simulink model "BEV_Thermal_Management"  (R2025a)
settings: Solver=ode23t  StartTime=0  StopTime=765  MaxStep=5  RelTol=1e-3  AbsTol=1e-3
model workspace: external: MATLAB File BEV_Thermal_Management_param.m (data not in the file)
undefined symbols (not defined in the file): Battery, bulb, cabin_doors_conductivity, cabin_duct_area, cabin_glass_conductivity, cabin_roof_conductivity, cabin_T_init, chiller_area_primary, chiller_N_baffles, chiller_N_tubes, chiller_tube_D, chiller_tube_L, chiller_wall_conductivity, chiller_wall_thickness, compressor_rpm_LUT, condenser_air_area_flow, condenser_air_area_primary, condenser_W, condenser_wall_conductivity, condenser_wall_thickness, coolant_channel_D, coolant_pipe_area, coolant_pipe_D, coolant_T_init, coolant_tank_area, coolant_tank_volume, coolant_valve_D_ratio_max, coolant_valve_D_ratio_min, coolant_valve_displacement, coolant_valve_S_max, cycle, DCDC, Edrive, evaporator_air_area_flow, evaporator_air_area_primary, evaporator_W, evaporator_wall_conductivity, evaporator_wall_thickness, heater_max_power, ModuleType1, outlet, ptc_max_power, pump_speed_max, radiationReflectionShields, radiator_air_area_flow, radiator_air_area_primary, radiator_W, radiator_wall_conductivity, radiator_wall_thickness, refrigerant_alpha_init, refrigerant_pipe_D, transRatio
libraries: fl_lib x264, nesl_utility x91, SimscapeFluids_lib x22, sdl_lib x13, ee_lib x9, nesl_utility_internal x4, slpidlib x3, BatteryProtection x3, batt_lib x2, BatteryCurrentManagement x1, autolibsharedcommon x1, simulink x1
(part 7 of 9)

== system BEV_Thermal_Management/Chiller/SR4 ==
  Absolute Reference (2P) : fl_lib/Two-Phase Fluid/Elements/Absolute Reference (2P)
  Mass & Energy Flow Rate Sensor (2P) : fl_lib/Two-Phase Fluid/Sensors/Flow Rate Sensor (2P)  mass_flow_measure=true  volumetric_flow_measure=false  energy_flow_measure=true
      settings: InternalSimscapePortConfiguration="{\"Bottom\":[{\"id\":\"PHI\",\"label\":\"φ\",\"type\":\"output\"}],\"Left\":[{\"id\":\"A\",\"label\":\"A\",\"type\":\"foundation.two_phase_fluid.two_phase_fluid\"}],\"Right\":[{\"id\":\"B\",\"label\":\"B\",\"type\":\"foundation.two_phase_fluid.two_phase_fluid\"},{\"id\":\"M\",\"label\":\"M\",\"type\":\"output\"}],\"Top\":[]}"
  PS-Simulink Converter : nesl_utility/PS-Simulink Converter  PhysicalDomain=network_engine_domain  SubClassName=ps_output  LeftPortType=input  RightPortType=output  PseudoPeriodic=off  Frequencies=[]  VectorFormat=1-D array  Unit=W  AffineConversion=off
  PS-Simulink Converter1 : nesl_utility/PS-Simulink Converter  PhysicalDomain=network_engine_domain  SubClassName=ps_output  LeftPortType=input  RightPortType=output  PseudoPeriodic=off  Frequencies=[]  VectorFormat=1-D array  Unit=MPa  AffineConversion=off
  PS-Simulink Converter2 : nesl_utility/PS-Simulink Converter  PhysicalDomain=network_engine_domain  SubClassName=ps_output  LeftPortType=input  RightPortType=output  PseudoPeriodic=off  Frequencies=[]  VectorFormat=inherit  Unit=degC  AffineConversion=off
  Pressure & Internal Energy Sensor (2P) : fl_lib/Two-Phase Fluid/Sensors/Pressure, Temperature & Internal Energy Sensor (2P)  reference=foundation.enum.MeasurementReference.difference  pressure=true  pressure_spec=foundation.enum.PressureMeasementSpec.Absolute  temperature=false  internal_energy=true
      settings: InternalSimscapePortConfiguration="{\"Bottom\":[{\"id\":\"U\",\"label\":\"U\",\"type\":\"output\"}],\"Left\":[{\"id\":\"A\",\"label\":\"A\",\"type\":\"foundation.two_phase_fluid.two_phase_fluid\"}],\"Right\":[{\"id\":\"B\",\"label\":\"B\",\"type\":\"foundation.two_phase_fluid.two_phase_fluid\"},{\"id\":\"P\",\"label\":\"P\",\"type\":\"output\"}],\"Top\":[]}"
  Terminator : Terminator
  Thermodynamic Properties Sensor (2P)1 : fl_lib/Two-Phase Fluid/Sensors/Thermodynamic Properties Sensor (2P)  temperature=true  enthalpy=true  density=false  specific_volume=true  entropy=true
      settings: InternalSimscapePortConfiguration="{\"Bottom\":[{\"id\":\"V\",\"label\":\"v\",\"type\":\"output\"},{\"id\":\"S\",\"label\":\"s\",\"type\":\"output\"}],\"Left\":[{\"id\":\"A\",\"label\":\"A\",\"type\":\"foundation.two_phase_fluid.two_phase_fluid\"}],\"Right\":[{\"id\":\"T\",\"label\":\"T\",\"type\":\"output\"},{\"id\":\"H\",\"label\":\"h\",\"type\":\"output\"}],\"Top\":[]}"
  B : PMIOPort  Side=Left
  A : PMIOPort  Port=2  Side=Right
  tag scope: Phi_chiller_out=global, p_chiller=global
  wires:
  PS-Simulink Converter/1 -> [Phi_chiller_out]
  PS-Simulink Converter1/1 -> [p_chiller]
  PS-Simulink Converter2/1 -> Terminator/1  "tempRefChillOut"
  connections:
  B/RConn1 -- Mass & Energy Flow Rate Sensor (2P)/RConn1
  Mass & Energy Flow Rate Sensor (2P)/LConn1 -- Thermodynamic Properties Sensor (2P)1/LConn1 -- Pressure & Internal Energy Sensor (2P)/LConn1 -- A/RConn1
  Mass & Energy Flow Rate Sensor (2P)/RConn3 -- PS-Simulink Converter/LConn1
  Absolute Reference (2P)/LConn1 -- Pressure & Internal Energy Sensor (2P)/RConn1
  PS-Simulink Converter1/LConn1 -- Pressure & Internal Energy Sensor (2P)/RConn2
  PS-Simulink Converter2/LConn1 -- Thermodynamic Properties Sensor (2P)1/RConn1

== system BEV_Thermal_Management/Compressor/Power sensor ==
  MRR3 : fl_lib/Mechanical/Rotational Elements/Mechanical Rotational Reference
  Pump power : fl_lib/Physical Signals/Functions/PS Product
  Rotational Motion Sensor : fl_lib/Mechanical/Mechanical Sensors/Ideal Rotational Motion Sensor  reference=foundation.enum.MeasurementReference.difference  acceleration_port=false  velocity_port=true  position_port=true  wrap_angle=simscape.enum.onoff.off  offset=0 rad
  Torque Sensor : fl_lib/Mechanical/Mechanical Sensors/Ideal Torque Sensor
  A : PMIOPort  Side=Left
  P : PMIOPort  Port=2  Side=Left
  B : PMIOPort  Port=3  Side=Right
  connections:
  Torque Sensor/RConn2 -- Pump power/LConn1
  Torque Sensor/RConn1 -- B/RConn1
  Rotational Motion Sensor/LConn1 -- Torque Sensor/LConn1 -- A/RConn1
  Rotational Motion Sensor/RConn2 -- Pump power/LConn2
  MRR3/LConn1 -- Rotational Motion Sensor/RConn1
  Pump power/RConn1 -- P/RConn1

== system BEV_Thermal_Management/Condenser/Power sensor ==
  MRR3 : fl_lib/Mechanical/Rotational Elements/Mechanical Rotational Reference
  Pump power : fl_lib/Physical Signals/Functions/PS Product
  Rotational Motion Sensor : fl_lib/Mechanical/Mechanical Sensors/Ideal Rotational Motion Sensor  reference=foundation.enum.MeasurementReference.difference  acceleration_port=false  velocity_port=true  position_port=true  wrap_angle=simscape.enum.onoff.off  offset=0 rad
  Torque Sensor : fl_lib/Mechanical/Mechanical Sensors/Ideal Torque Sensor
  A : PMIOPort  Side=Left
  P : PMIOPort  Port=2  Side=Left
  B : PMIOPort  Port=3  Side=Right
  connections:
  Torque Sensor/RConn2 -- Pump power/LConn1
  Torque Sensor/RConn1 -- B/RConn1
  Rotational Motion Sensor/LConn1 -- Torque Sensor/LConn1 -- A/RConn1
  Rotational Motion Sensor/RConn2 -- Pump power/LConn2
  MRR3/LConn1 -- Rotational Motion Sensor/RConn1
  Pump power/RConn1 -- P/RConn1

== system BEV_Thermal_Management/Condenser/SR1 ==
  Absolute Reference (2P) : fl_lib/Two-Phase Fluid/Elements/Absolute Reference (2P)
  Mass & Energy Flow Rate Sensor (2P) : fl_lib/Two-Phase Fluid/Sensors/Flow Rate Sensor (2P)  mass_flow_measure=true  volumetric_flow_measure=false  energy_flow_measure=true
      settings: InternalSimscapePortConfiguration="{\"Bottom\":[{\"id\":\"PHI\",\"label\":\"φ\",\"type\":\"output\"}],\"Left\":[{\"id\":\"A\",\"label\":\"A\",\"type\":\"foundation.two_phase_fluid.two_phase_fluid\"}],\"Right\":[{\"id\":\"B\",\"label\":\"B\",\"type\":\"foundation.two_phase_fluid.two_phase_fluid\"},{\"id\":\"M\",\"label\":\"M\",\"type\":\"output\"}],\"Top\":[]}"
  PS-Simulink Converter : nesl_utility/PS-Simulink Converter  PhysicalDomain=network_engine_domain  SubClassName=ps_output  LeftPortType=input  RightPortType=output  PseudoPeriodic=off  Frequencies=[]  VectorFormat=1-D array  Unit=W  AffineConversion=off
  PS-Simulink Converter2 : nesl_utility/PS-Simulink Converter  PhysicalDomain=network_engine_domain  SubClassName=ps_output  LeftPortType=input  RightPortType=output  PseudoPeriodic=off  Frequencies=[]  VectorFormat=inherit  Unit=degC  AffineConversion=off
  Pressure & Internal Energy Sensor (2P) : fl_lib/Two-Phase Fluid/Sensors/Pressure, Temperature & Internal Energy Sensor (2P)  reference=foundation.enum.MeasurementReference.difference  pressure=true  pressure_spec=foundation.enum.PressureMeasementSpec.Absolute  temperature=false  internal_energy=true
      settings: InternalSimscapePortConfiguration="{\"Bottom\":[{\"id\":\"U\",\"label\":\"U\",\"type\":\"output\"}],\"Left\":[{\"id\":\"A\",\"label\":\"A\",\"type\":\"foundation.two_phase_fluid.two_phase_fluid\"}],\"Right\":[{\"id\":\"B\",\"label\":\"B\",\"type\":\"foundation.two_phase_fluid.two_phase_fluid\"},{\"id\":\"P\",\"label\":\"P\",\"type\":\"output\"}],\"Top\":[]}"
  Terminator : Terminator
  Thermodynamic Properties Sensor (2P) : fl_lib/Two-Phase Fluid/Sensors/Thermodynamic Properties Sensor (2P)  temperature=true  enthalpy=true  density=false  specific_volume=true  entropy=true
      settings: InternalSimscapePortConfiguration="{\"Bottom\":[{\"id\":\"V\",\"label\":\"v\",\"type\":\"output\"},{\"id\":\"S\",\"label\":\"s\",\"type\":\"output\"}],\"Left\":[{\"id\":\"A\",\"label\":\"A\",\"type\":\"foundation.two_phase_fluid.two_phase_fluid\"}],\"Right\":[{\"id\":\"T\",\"label\":\"T\",\"type\":\"output\"},{\"id\":\"H\",\"label\":\"h\",\"type\":\"output\"}],\"Top\":[]}"
  A : PMIOPort  Side=Left
  B : PMIOPort  Port=2  Side=Right
  tag scope: Phi_cond_in=global
  wires:
  PS-Simulink Converter/1 -> [Phi_cond_in]
  PS-Simulink Converter2/1 -> Terminator/1  "tempRefCondIn"
  connections:
  Mass & Energy Flow Rate Sensor (2P)/LConn1 -- Pressure & Internal Energy Sensor (2P)/LConn1 -- Thermodynamic Properties Sensor (2P)/LConn1 -- A/RConn1
  B/RConn1 -- Mass & Energy Flow Rate Sensor (2P)/RConn1
  PS-Simulink Converter/LConn1 -- Mass & Energy Flow Rate Sensor (2P)/RConn3
  Absolute Reference (2P)/LConn1 -- Pressure & Internal Energy Sensor (2P)/RConn1
  PS-Simulink Converter2/LConn1 -- Thermodynamic Properties Sensor (2P)/RConn1

== system BEV_Thermal_Management/Condenser/SR2 ==
  Absolute Reference (2P) : fl_lib/Two-Phase Fluid/Elements/Absolute Reference (2P)
  Mass & Energy Flow Rate Sensor (2P) : fl_lib/Two-Phase Fluid/Sensors/Flow Rate Sensor (2P)  mass_flow_measure=true  volumetric_flow_measure=false  energy_flow_measure=true
      settings: InternalSimscapePortConfiguration="{\"Bottom\":[{\"id\":\"PHI\",\"label\":\"φ\",\"type\":\"output\"}],\"Left\":[{\"id\":\"A\",\"label\":\"A\",\"type\":\"foundation.two_phase_fluid.two_phase_fluid\"}],\"Right\":[{\"id\":\"B\",\"label\":\"B\",\"type\":\"foundation.two_phase_fluid.two_phase_fluid\"},{\"id\":\"M\",\"label\":\"M\",\"type\":\"output\"}],\"Top\":[]}"
  PS-Simulink Converter : nesl_utility/PS-Simulink Converter  PhysicalDomain=network_engine_domain  SubClassName=ps_output  LeftPortType=input  RightPortType=output  PseudoPeriodic=off  Frequencies=[]  VectorFormat=1-D array  Unit=W  AffineConversion=off
  PS-Simulink Converter1 : nesl_utility/PS-Simulink Converter  PhysicalDomain=network_engine_domain  SubClassName=ps_output  LeftPortType=input  RightPortType=output  PseudoPeriodic=off  Frequencies=[]  VectorFormat=1-D array  Unit=MPa  AffineConversion=off
  PS-Simulink Converter2 : nesl_utility/PS-Simulink Converter  PhysicalDomain=network_engine_domain  SubClassName=ps_output  LeftPortType=input  RightPortType=output  PseudoPeriodic=off  Frequencies=[]  VectorFormat=inherit  Unit=degC  AffineConversion=off
  Pressure & Internal Energy Sensor (2P) : fl_lib/Two-Phase Fluid/Sensors/Pressure, Temperature & Internal Energy Sensor (2P)  reference=foundation.enum.MeasurementReference.difference  pressure=true  pressure_spec=foundation.enum.PressureMeasementSpec.Absolute  temperature=false  internal_energy=true
      settings: InternalSimscapePortConfiguration="{\"Bottom\":[{\"id\":\"U\",\"label\":\"U\",\"type\":\"output\"}],\"Left\":[{\"id\":\"A\",\"label\":\"A\",\"type\":\"foundation.two_phase_fluid.two_phase_fluid\"}],\"Right\":[{\"id\":\"B\",\"label\":\"B\",\"type\":\"foundation.two_phase_fluid.two_phase_fluid\"},{\"id\":\"P\",\"label\":\"P\",\"type\":\"output\"}],\"Top\":[]}"
  Terminator : Terminator
  Thermodynamic Properties Sensor (2P) : fl_lib/Two-Phase Fluid/Sensors/Thermodynamic Properties Sensor (2P)  temperature=true  enthalpy=true  density=false  specific_volume=true  entropy=true
      settings: InternalSimscapePortConfiguration="{\"Bottom\":[{\"id\":\"V\",\"label\":\"v\",\"type\":\"output\"},{\"id\":\"S\",\"label\":\"s\",\"type\":\"output\"}],\"Left\":[{\"id\":\"A\",\"label\":\"A\",\"type\":\"foundation.two_phase_fluid.two_phase_fluid\"}],\"Right\":[{\"id\":\"T\",\"label\":\"T\",\"type\":\"output\"},{\"id\":\"H\",\"label\":\"h\",\"type\":\"output\"}],\"Top\":[]}"
  A : PMIOPort  Side=Left
  B : PMIOPort  Port=2  Side=Right
  tag scope: Phi_cond_out=global, p_cond=global
  wires:
  PS-Simulink Converter/1 -> [Phi_cond_out]
  PS-Simulink Converter1/1 -> [p_cond]
  PS-Simulink Converter2/1 -> Terminator/1  "tempRefCondOut"
  connections:
  Mass & Energy Flow Rate Sensor (2P)/LConn1 -- Thermodynamic Properties Sensor (2P)/LConn1 -- Pressure & Internal Energy Sensor (2P)/LConn1 -- A/RConn1
  B/RConn1 -- Mass & Energy Flow Rate Sensor (2P)/RConn1
  PS-Simulink Converter/LConn1 -- Mass & Energy Flow Rate Sensor (2P)/RConn3
  Absolute Reference (2P)/LConn1 -- Pressure & Internal Energy Sensor (2P)/RConn1
  PS-Simulink Converter1/LConn1 -- Pressure & Internal Energy Sensor (2P)/RConn2
  PS-Simulink Converter2/LConn1 -- Thermodynamic Properties Sensor (2P)/RConn1

== system BEV_Thermal_Management/Condenser/Speed command ==
  Max Speed [rpm] : Gain  Gain=1100
  Transfer Fcn : TransferFcn  Denominator=[5 1]
  Out1 : Outport
  wires:
  Transfer Fcn/1 -> Max Speed [rpm]/1
  Max Speed [rpm]/1 -> Out1/1
  [cmd_fan] -> Transfer Fcn/1

== system BEV_Thermal_Management/Controls/Cabin Air Control ==
  note: if the outside temperature is higher then the setpoint temperature turn off the PTC
  T_cabin : Inport
  T_setpoint : Inport  Port=2
  T_env : Inport  Port=3
  T_ptc : Inport  Port=4
  Add : Sum  Inputs=-+
  Constant : Constant  Commented=on  Value=0
  Constant1 : Constant  Value=0
  Old cmd ptc : Terminator  Commented=on
  PID Controller : slpidlib/PID Controller  Controller=PI  Form=Ideal  TimeDomain=Continuous-time  UseExternalTs=off  SampleTime=-1  IntegratorMethod=Forward Euler  FilterMethod=Forward Euler  ControllerParametersSource=internal  P=1/50  I=1/150  UseKiTs=off  D=0  UseExternalDerivativeSource=off  N=100  UseFilter=on  TunerSelectOption=Transfer Function Based (PID Tuner App)  InitialConditionSource=internal  InitialConditionForIntegrator=0  InitialConditionForFilter=0  DifferentiatorICPrevScaledInput=0  ExternalReset=none  TrackingMode=off  Kt=1  LimitOutput=on  SatLimitsSource=internal  UpperSaturationLimit=1  LowerSaturationLimit=0  LinearizeAsGain=on  AntiWindupMode=back-calculation  Kb=1  LimitIntegrator=off  UpperIntegratorSaturationLimit=inf  LowerIntegratorSaturationLimit=-inf  POutMin=[]  POutMax=[]  IOutMin=[]  IOutMax=[]  DOutMin=[]  DOutMax=[]  NOutMin=[]  NOutMax=[]  SumOutMin=[]  SumOutMax=[]  SaturationOutMin=[]  SaturationOutMax=[]  PParamMin=[]  PParamMax=[]  IParamMin=[]  IParamMax=[]  DParamMin=[]  DParamMax=[]  NParamMin=[]  NParamMax=[]  KbParamMin=[]  KbParamMax=[]  KtParamMin=[]  KtParamMax=[]  KbOutMin=[]  KbOutMax=[]  KtOutMin=[]  KtOutMax=[]  IntegratorOutMin=[]  IntegratorOutMax=[]  FilterOutMin=[]  FilterOutMax=[]  SumI1OutMin=[]  SumI1OutMax=[]  SumI2OutMin=[]  SumI2OutMax=[]  SumI3OutMin=[]  SumI3OutMax=[]  SumI4OutMin=[]  SumI4OutMax=[]  SumDOutMin=[]  SumDOutMax=[]  DifferentiatorOutMin=[]  DifferentiatorOutMax=[]  FilterDiffOutCoefMin=[]  FilterDiffOutCoefMax=[]  ReciprocalOutMin=[]  ReciprocalOutMax=[]  SumDenOutMin=[]  SumDenOutMax=[]  SumNumOutMin=[]  SumNumOutMax=[]  DivideOutMin=[]  DivideOutMax=[]  UdiffTsProdOutMin=[]  UdiffTsProdOutMax=[]  NTsProdOutMin=[]  NTsProdOutMax=[]  UintegralTsProdOutMin=[]  UintegralTsProdOutMax=[]  UngainTsProdOutMin=[]  UngainTsProdOutMax=[]  ClampingZeroOutDataTypeStr=Inherit: Inherit via back propagation  ClampingZeroOutMin=[]  ClampingZeroOutMax=[]  FilterDenConstantOutDataTypeStr=Inherit: Inherit via back propagation  FilterDenConstantOutMin=[]  FilterDenConstantOutMax=[]  PCopyOutDataTypeStr=Inherit: Inherit via back propagation  PCopyOutMin=[]  PCopyOutMax=[]  NCopyOutDataTypeStr=Inherit: Inherit via back propagation  NCopyOutMin=[]  NCopyOutMax=[]  IntegratorContinuousStateAttributes=''  IntegratorStateMustResolveToSignalObject=off  IntegratorRTWStateStorageClass=Auto  FilterContinuousStateAttributes=''  FilterStateMustResolveToSignalObject=off  FilterRTWStateStorageClass=Auto  ParallelPVariant=Passthrough  IdealPVariant=InternalParameters  IVariant=InternalParameters  DVariant=Disabled  IntegratorVariant=Continuous  SatVariant=Enabled  AWVariant=BackCalculation  PCopyVariant=Disabled  TRVariant=Disabled  FdbkBlocksVariant=Forward  IdealPFdbkVariant=Disabled  SatFdbkVariant=Disabled  DerivativeFilterVariant=Disabled  NVariant=Disabled  NCopyVariant=Disabled_SignalSpec  FilterICVariant=Disabled  IntegratorICVariant=InternalICs  ExternalResetVariant=Disabled  TRSumVariant=Passthrough  SumFdbkVariant=Disabled  SumVariant=Sum_PI  TsampFilterVariant=InternalTs  TsampNgainVariant=Passthrough  TsampIntegralVariant=Disabled_SignalSpec  ExternalSaturationOutDataTypeStr=Inherit: Same as second input  DerivativeSourceVariant=Disabled  PreIntVariant=InternalPreInt
  PID Controller1 : slpidlib/PID Controller  Controller=PI  Form=Parallel  TimeDomain=Continuous-time  UseExternalTs=off  SampleTime=-1  IntegratorMethod=Forward Euler  FilterMethod=Forward Euler  ControllerParametersSource=internal  P=0.07  I=1e-5  UseKiTs=off  D=0  UseExternalDerivativeSource=off  N=100  UseFilter=on  TunerSelectOption=Transfer Function Based (PID Tuner App)  InitialConditionSource=internal  InitialConditionForIntegrator=0  InitialConditionForFilter=0  DifferentiatorICPrevScaledInput=0  ExternalReset=none  TrackingMode=off  Kt=1  LimitOutput=on  SatLimitsSource=internal  UpperSaturationLimit=1  LowerSaturationLimit=0  LinearizeAsGain=on  AntiWindupMode=none  Kb=1  LimitIntegrator=off  UpperIntegratorSaturationLimit=inf  LowerIntegratorSaturationLimit=-inf  POutMin=[]  POutMax=[]  IOutMin=[]  IOutMax=[]  DOutMin=[]  DOutMax=[]  NOutMin=[]  NOutMax=[]  SumOutMin=[]  SumOutMax=[]  SaturationOutMin=[]  SaturationOutMax=[]  PParamMin=[]  PParamMax=[]  IParamMin=[]  IParamMax=[]  DParamMin=[]  DParamMax=[]  NParamMin=[]  NParamMax=[]  KbParamMin=[]  KbParamMax=[]  KtParamMin=[]  KtParamMax=[]  KbOutMin=[]  KbOutMax=[]  KtOutMin=[]  KtOutMax=[]  IntegratorOutMin=[]  IntegratorOutMax=[]  FilterOutMin=[]  FilterOutMax=[]  SumI1OutMin=[]  SumI1OutMax=[]  SumI2OutMin=[]  SumI2OutMax=[]  SumI3OutMin=[]  SumI3OutMax=[]  SumI4OutMin=[]  SumI4OutMax=[]  SumDOutMin=[]  SumDOutMax=[]  DifferentiatorOutMin=[]  DifferentiatorOutMax=[]  FilterDiffOutCoefMin=[]  FilterDiffOutCoefMax=[]  ReciprocalOutMin=[]  ReciprocalOutMax=[]  SumDenOutMin=[]  SumDenOutMax=[]  SumNumOutMin=[]  SumNumOutMax=[]  DivideOutMin=[]  DivideOutMax=[]  UdiffTsProdOutMin=[]  UdiffTsProdOutMax=[]  NTsProdOutMin=[]  NTsProdOutMax=[]  UintegralTsProdOutMin=[]  UintegralTsProdOutMax=[]  UngainTsProdOutMin=[]  UngainTsProdOutMax=[]  ClampingZeroOutDataTypeStr=Inherit: Inherit via back propagation  ClampingZeroOutMin=[]  ClampingZeroOutMax=[]  FilterDenConstantOutDataTypeStr=Inherit: Inherit via back propagation  FilterDenConstantOutMin=[]  FilterDenConstantOutMax=[]  PCopyOutDataTypeStr=Inherit: Inherit via back propagation  PCopyOutMin=[]  PCopyOutMax=[]  NCopyOutDataTypeStr=Inherit: Inherit via back propagation  NCopyOutMin=[]  NCopyOutMax=[]  IntegratorContinuousStateAttributes=''  IntegratorStateMustResolveToSignalObject=off  IntegratorRTWStateStorageClass=Auto  FilterContinuousStateAttributes=''  FilterStateMustResolveToSignalObject=off  FilterRTWStateStorageClass=Auto  ParallelPVariant=InternalParameters  IdealPVariant=Disabled  IVariant=InternalParameters  DVariant=Disabled  IntegratorVariant=Continuous  SatVariant=Enabled  AWVariant=Passthrough  PCopyVariant=Disabled  TRVariant=Disabled  FdbkBlocksVariant=Forward  IdealPFdbkVariant=Disabled  SatFdbkVariant=Disabled  DerivativeFilterVariant=Disabled  NVariant=Disabled  NCopyVariant=Disabled_SignalSpec  FilterICVariant=Disabled  IntegratorICVariant=InternalICs  ExternalResetVariant=Disabled  TRSumVariant=Passthrough  SumFdbkVariant=Disabled  SumVariant=Sum_PI  TsampFilterVariant=InternalTs  TsampNgainVariant=Passthrough  TsampIntegralVariant=Disabled_SignalSpec  ExternalSaturationOutDataTypeStr=Inherit: Same as second input  DerivativeSourceVariant=Disabled  PreIntVariant=InternalPreInt
  Product : Product
  Relay : Relay  Commented=on  OnSwitchValue=45  OffSwitchValue=35  OnOutputValue=0  OffOutputValue=1  ZeroCross=off
  Sign : Signum
  Sum : Sum  Inputs=-+|
  Sum1 : Sum  Inputs=-+|
  Switch : Switch  Commented=on  SaturateOnIntegerOverflow=off  InputSameDT=off
  Switch1 : Switch  Criteria=u2 > Threshold  SaturateOnIntegerOverflow=off  InputSameDT=off
  Target Temp Out : Constant  Value=40
  cmd_blower : Outport
  cmd_ptc : Outport  Port=2
  wires:
  T_setpoint/1 -> Sum1/1, Sum/1
  Sum1/1 -> Switch/2, Switch1/2, Sign/1
  Product/1 -> PID Controller/1
  PID Controller/1 -> cmd_blower/1
  T_env/1 -> Sum1/2
  Sum/1 -> Product/1
  Sign/1 -> Product/2
  Constant/1 -> Switch/1
  Relay/1 -> Switch/3
  T_ptc/1 -> Relay/1, Add/1
  T_cabin/1 -> Sum/2
  Switch/1 -> Old cmd ptc/1
  Add/1 -> PID Controller1/1
  Target Temp Out/1 -> Add/2
  Constant1/1 -> Switch1/1
  PID Controller1/1 -> Switch1/3
  Switch1/1 -> cmd_ptc/1

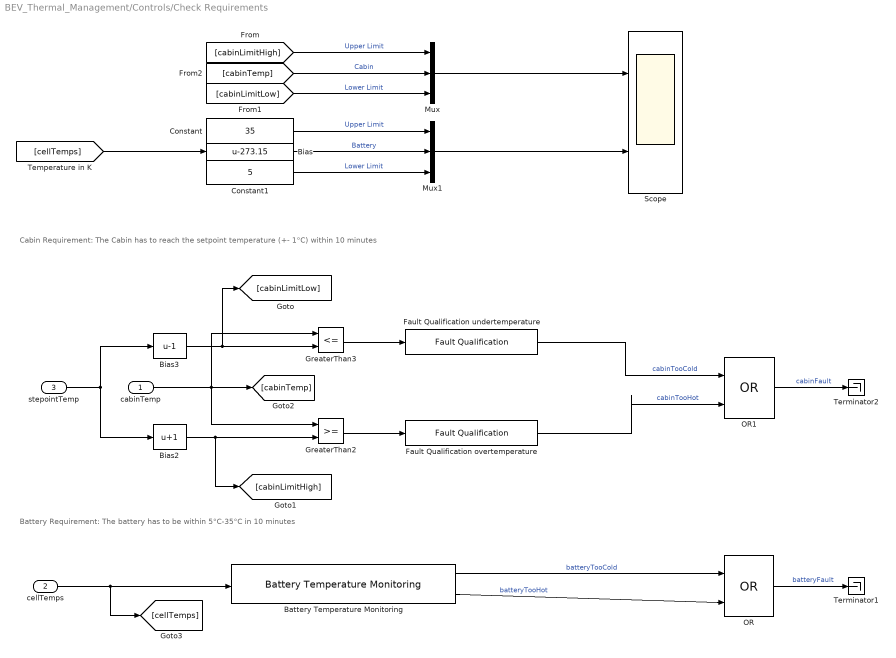
== system BEV_Thermal_Management/Controls/Check Requirements ==
  note: Cabin Requirement: The Cabin has to reach the setpoint temperature (+- 1°C) within 10 minutes
  note: Battery Requirement: The battery has to be within 5°C-35°C in 10 minutes
  cabinTemp : Inport
  cellTemps : Inport  Port=2
  stepointTemp : Inport  Port=3
  Battery Temperature Monitoring : BatteryProtection/Battery Temperature Monitoring  MinMaxFlag=off  UndertemperatureLimit=5+273.15  OvertemperatureLimit=35+273.15  QualTimeUndertemp=600  DisqualTimeUndertemp=0  QualTimeOvertemp=600  DisqualTimeOvertemp=0  Ts=-1  DataType=Inherit: auto
      settings: LibrarySourceBlock=|
      | batt_sl_lib/Protection/Battery Temperature
      | Monitoring
  Bias : Bias  Bias=-273.15  SaturateOnIntegerOverflow=off
  Bias2 : Bias  Bias=1  SaturateOnIntegerOverflow=off
  Bias3 : Bias  Bias=-1  SaturateOnIntegerOverflow=off
  Constant : Constant  Value=35
  Constant1 : Constant  Value=5
  Fault Qualification overtemperature : BatteryProtection/Fault Qualification  QualTime=600  DisqualTime=0  Ts=-1
      settings: LibrarySourceBlock=|
      | BatteryProtection/Battery Temperature
      | Monitoring/Fault Qualification overtemperature
  Fault Qualification undertemperature : BatteryProtection/Fault Qualification  QualTime=600  DisqualTime=0  Ts=-1
      settings: LibrarySourceBlock=|
      | BatteryProtection/Battery Temperature
      | Monitoring/Fault Qualification undertemperature
  GreaterThan2 : RelationalOperator  OutDataTypeStr=boolean  RndMeth=Simplest  InputSameDT=off
  GreaterThan3 : RelationalOperator  Operator=<=  OutDataTypeStr=boolean  RndMeth=Simplest  InputSameDT=off
  Mux : Mux  Inputs=3
  Mux1 : Mux  Inputs=3
  OR : Logic  Operator=OR  IconShape=distinctive  AllPortsSameDT=off  OutDataTypeStr=boolean
  OR1 : Logic  Operator=OR  IconShape=distinctive  AllPortsSameDT=off  OutDataTypeStr=boolean
  Scope : Scope  NumInputPorts=2
      settings: ActiveDisplayYMinimum=21.9941  ActiveDisplayYMaximum=42.05306
  Terminator1 : Terminator
  Terminator2 : Terminator
  wires:
  cellTemps/1 -> [cellTemps], Battery Temperature Monitoring/1
  OR/1 -> Terminator1/1  "batteryFault"
  Battery Temperature Monitoring/1 -> OR/1  "batteryTooCold"
  Battery Temperature Monitoring/2 -> OR/2  "batteryTooHot"
  GreaterThan2/1 -> Fault Qualification overtemperature/1
  cabinTemp/1 -> [cabinTemp], GreaterThan3/1, GreaterThan2/1
  GreaterThan3/1 -> Fault Qualification undertemperature/1
  Bias2/1 -> [cabinLimitHigh], GreaterThan2/2
  stepointTemp/1 -> Bias3/1, Bias2/1
  Bias3/1 -> [cabinLimitLow], GreaterThan3/2
  Fault Qualification undertemperature/1 -> OR1/1  "cabinTooCold"
  Fault Qualification overtemperature/1 -> OR1/2  "cabinTooHot"
  OR1/1 -> Terminator2/1  "cabinFault"
  [cabinLimitHigh] -> Mux/1  "Upper Limit"
  [cabinLimitLow] -> Mux/3  "Lower Limit"
  [cabinTemp] -> Mux/2  "Cabin"
  Mux/1 -> Scope/1
  Mux1/1 -> Scope/2
  Constant/1 -> Mux1/1  "Upper Limit"
  Constant1/1 -> Mux1/3  "Lower Limit"
  [cellTemps] -> Bias/1
  Bias/1 -> Mux1/2  "Battery"

== system BEV_Thermal_Management/Controls/Compressor Control ==
  p_evap : Inport
  p_chiller : Inport  Port=2
  cmd_chiller_bypass : Inport  Port=3
  ac_onoff : Inport  Port=4
  Constant : Constant
  Constant1 : Constant  Value=0
  Freezing Cutoff : Lookup_n-D  NumberOfTableDimensions=1  BreakpointsForDimension1=[0 0.15 0.25 0.4]  IndexSearchMethod=Linear search  BeginIndexSearchUsingPreviousIndexResult=on  Table=[0 0 1 1]  InternalRulePriority=Speed  RndMeth=Simplest
  MinMax : MinMax  Function=max  Inputs=2  ZeroCross=off
  MinMax1 : MinMax  Inputs=2  ZeroCross=off
  MinMax2 : MinMax  Function=max  Inputs=2
  PID Controller : slpidlib/PID Controller  Controller=PI  Form=Ideal  TimeDomain=Continuous-time  UseExternalTs=off  SampleTime=-1  IntegratorMethod=Forward Euler  FilterMethod=Forward Euler  ControllerParametersSource=internal  P=1%1  I=1/5  UseKiTs=off  D=0  UseExternalDerivativeSource=off  N=100  UseFilter=on  TunerSelectOption=Transfer Function Based (PID Tuner App)  InitialConditionSource=internal  InitialConditionForIntegrator=0  InitialConditionForFilter=0  DifferentiatorICPrevScaledInput=0  ExternalReset=none  TrackingMode=off  Kt=1  LimitOutput=on  SatLimitsSource=internal  UpperSaturationLimit=1  LowerSaturationLimit=0  LinearizeAsGain=on  AntiWindupMode=back-calculation  Kb=1  LimitIntegrator=off  UpperIntegratorSaturationLimit=inf  LowerIntegratorSaturationLimit=-inf  POutMin=[]  POutMax=[]  IOutMin=[]  IOutMax=[]  DOutMin=[]  DOutMax=[]  NOutMin=[]  NOutMax=[]  SumOutMin=[]  SumOutMax=[]  SaturationOutMin=[]  SaturationOutMax=[]  PParamMin=[]  PParamMax=[]  IParamMin=[]  IParamMax=[]  DParamMin=[]  DParamMax=[]  NParamMin=[]  NParamMax=[]  KbParamMin=[]  KbParamMax=[]  KtParamMin=[]  KtParamMax=[]  KbOutMin=[]  KbOutMax=[]  KtOutMin=[]  KtOutMax=[]  IntegratorOutMin=[]  IntegratorOutMax=[]  FilterOutMin=[]  FilterOutMax=[]  SumI1OutMin=[]  SumI1OutMax=[]  SumI2OutMin=[]  SumI2OutMax=[]  SumI3OutMin=[]  SumI3OutMax=[]  SumI4OutMin=[]  SumI4OutMax=[]  SumDOutMin=[]  SumDOutMax=[]  DifferentiatorOutMin=[]  DifferentiatorOutMax=[]  FilterDiffOutCoefMin=[]  FilterDiffOutCoefMax=[]  ReciprocalOutMin=[]  ReciprocalOutMax=[]  SumDenOutMin=[]  SumDenOutMax=[]  SumNumOutMin=[]  SumNumOutMax=[]  DivideOutMin=[]  DivideOutMax=[]  UdiffTsProdOutMin=[]  UdiffTsProdOutMax=[]  NTsProdOutMin=[]  NTsProdOutMax=[]  UintegralTsProdOutMin=[]  UintegralTsProdOutMax=[]  UngainTsProdOutMin=[]  UngainTsProdOutMax=[]  ClampingZeroOutDataTypeStr=Inherit: Inherit via back propagation  ClampingZeroOutMin=[]  ClampingZeroOutMax=[]  FilterDenConstantOutDataTypeStr=Inherit: Inherit via back propagation  FilterDenConstantOutMin=[]  FilterDenConstantOutMax=[]  PCopyOutDataTypeStr=Inherit: Inherit via back propagation  PCopyOutMin=[]  PCopyOutMax=[]  NCopyOutDataTypeStr=Inherit: Inherit via back propagation  NCopyOutMin=[]  NCopyOutMax=[]  IntegratorContinuousStateAttributes=''  IntegratorStateMustResolveToSignalObject=off  IntegratorRTWStateStorageClass=Auto  FilterContinuousStateAttributes=''  FilterStateMustResolveToSignalObject=off  FilterRTWStateStorageClass=Auto  ParallelPVariant=Passthrough  IdealPVariant=InternalParameters  IVariant=InternalParameters  DVariant=Disabled  IntegratorVariant=Continuous  SatVariant=Enabled  AWVariant=BackCalculation  PCopyVariant=Disabled  TRVariant=Disabled  FdbkBlocksVariant=Forward  IdealPFdbkVariant=Disabled  SatFdbkVariant=Disabled  DerivativeFilterVariant=Disabled  NVariant=Disabled  NCopyVariant=Disabled_SignalSpec  FilterICVariant=Disabled  IntegratorICVariant=InternalICs  ExternalResetVariant=Disabled  TRSumVariant=Passthrough  SumFdbkVariant=Disabled  SumVariant=Sum_PI  TsampFilterVariant=InternalTs  TsampNgainVariant=Passthrough  TsampIntegralVariant=Disabled_SignalSpec  ExternalSaturationOutDataTypeStr=Inherit: Same as second input  DerivativeSourceVariant=Disabled  PreIntVariant=InternalPreInt
  Pressure Target [MPa] : Constant  Value=0.3
  Product : Product
  Sum : Sum  Inputs=+-|
  Sum1 : Sum  Inputs=-+|
  Switch : Switch  Criteria=u2 > Threshold  Threshold=0.5  SaturateOnIntegerOverflow=off  InputSameDT=off
  cmd_comp : Outport
  wires:
  cmd_chiller_bypass/1 -> Sum/2
  Constant/1 -> Sum/1
  Sum/1 -> MinMax2/1
  ac_onoff/1 -> MinMax2/2
  Switch/1 -> cmd_comp/1
  Sum1/1 -> PID Controller/1
  MinMax2/1 -> Switch/2
  Product/1 -> Switch/1
  PID Controller/1 -> Product/1
  MinMax1/1 -> Freezing Cutoff/1
  Freezing Cutoff/1 -> Product/2
  p_chiller/1 -> MinMax1/2, MinMax/2
  Constant1/1 -> Switch/3
  Pressure Target [MPa]/1 -> Sum1/1
  p_evap/1 -> MinMax/1, MinMax1/1
  MinMax/1 -> Sum1/2

== system BEV_Thermal_Management/Controls/Coolant Loop Control ==
  note: Modified so that the parallel mode is not activated in winter
  note: Modified so that it does not activate too early
  note: I had to change the heater to use the temperature of the battery otherwise it would not heat at all
  T_env : Inport
  T_coolant_battery_in : Inport  Port=2
  T_motor : Inport  Port=3
  T_battery : Inport  Port=4
  T_coolant_inverter_out : Inport  Port=5
  Battery Heater : Subsystem
  Battery Pump : Subsystem
  Chiller Bypass : Subsystem
  Motor Pump : Subsystem
  Parallel-Serial Mode : Subsystem
  Radiator Bypass : Subsystem
  Terminator : Terminator
  cmd_heater : Outport
  cmd_motor_pump : Outport  Port=2
  cmd_battery_pump : Outport  Port=3
  cmd_chiller_bypass : Outport  Port=4
  cmd_parallel_serial : Outport  Port=5
  cmd_rad_bypass : Outport  Port=6
  wires:
  Parallel-Serial Mode/1(cmd_parallel_serial) -> cmd_parallel_serial/1, Battery Pump/4(parallel_serial)
  Motor Pump/1(cmd_motor_pump) -> Battery Pump/1(cmd_motor_pump), cmd_motor_pump/1
  T_env/1 -> Battery Heater/1(T_env), Parallel-Serial Mode/2(T_env)
  T_coolant_inverter_out/1 -> Parallel-Serial Mode/3(T_coolant_inverter_out), Radiator Bypass/1(T_coolant_inverter_out)
  T_motor/1 -> Motor Pump/1(T_motor)
  Battery Heater/1(cmd_heater) -> cmd_heater/1
  Battery Pump/1(cmd_battery_pump) -> cmd_battery_pump/1
  Radiator Bypass/1(cmd_rad_bypass) -> cmd_rad_bypass/1
  Chiller Bypass/1(cmd_chiller_bypass) -> Battery Pump/3(cmd_chiller_bypass), Parallel-Serial Mode/1(cmd_chiller_bypass), cmd_chiller_bypass/1
  T_battery/1 -> Battery Heater/2(T_coolant_battery_in), Chiller Bypass/1(T_battery), Battery Pump/2(T_battery)
  T_coolant_battery_in/1 -> Terminator/1

== system BEV_Thermal_Management/Controls/Driver and Regen ==
  EMSpd : Inport
  VehSpdFdbk : Inport  Port=2
  VehRef : Inport  Port=3
  Constant : Constant  Value=0
  Longitudinal Driver : Subsystem  SystemSampleTime=.01  mask(Longitudinal Driver){extAccelOvr=off, extDecelOvr=off, extAccelHld=off, extDecelHld=off, extAccelZero=off, extDecelZero=off, cntrlType=Predictive, shftType=None, velUnits=km/hr, gearOut=off, Kp=10, Ki=5, Kff=.1, Kg=0, VehVelVec=[0 100], KffVec=[.1 .1], KpVec=[10 10], KiVec=[5 5], KgVec=[0 0], m=1623, Kpt=16000, tau=0.08, L=4, aR=200, bR=2.5, cR=0.5, g=9.8, vnom=5, Kaw=1, tauerr=.01, tauPt=2, GearInit=0, tShift=0.1, pdlVec=[0.1 0.4 0.5 0.9], upShftTbl=[-1 12.9375 26.4375 39.9375 51.18749999999999 62.4375 72.84375 83.25;-1 16.3125 29.8125 43.3125 54.5624 65.8125 76.78125 87.75;-1 19.6875 33.1875 46.68749999999999 57.9375 69.1875 80.71875 92.25;-1 33 52.5 77.25 100.5 138.75 161.875 185], dwnShftTbl=[1 9.5625 23.0625 36.5625 47.8125 59.0625 68.90625 78.75;1 12.9375 26.4375 39.9375 51.18749999999999 62.4375 72.84375 83.25;1 16.3125 29.8125 43.3125 54.562499 65.8125 76.78125 87.75;1 19.6875 33.1875 46.68749999999999 57.9375 69.1875 80.71875 92.25], tClutch=.5, tRev=.5, tPark=120, aMode=6, UpGearVec=[0  1  2  3  4  5  6  7], DownGearVec=[1  2  3  4  5  6  7  8]}
      mask prompts: extAccelOvr "autoblks_shared:autoblkLongitudinalDriver:blkPrm_extAccelOvr"; extDecelOvr "autoblks_shared:autoblkLongitudinalDriver:blkPrm_extDeccelOvr"; extAccelHld "autoblks_shared:autoblkLongitudinalDriver:blkPrm_extAccelHld"; extDecelHld "autoblks_shared:autoblkLongitudinalDriver:blkPrm_extDeccelHld"; extAccelZero "autoblks_shared:autoblkLongitudinalDriver:blkPrm_extAccelZero"; extDecelZero "autoblks_shared:autoblkLongitudinalDriver:blkPrm_extDeccelZero"; cntrlType "autoblks_shared:autoblkLongitudinalDriver:blkPrm_cntrlType"; shftType "autoblks_shared:autoblkLongitudinalDriver:blkPrm_shftType"; velUnits "autoblks_shared:autoblkLongitudinalDriver:blkPrm_velUnits"; gearOut "autoblks_shared:autoblkLongitudinalDriver:blkPrm_gearOut"; Kp "autoblks_shared:autoblkLongitudinalDriver:blkPrm_Kp"; Ki "autoblks_shared:autoblkLongitudinalDriver:blkPrm_Ki"; Kff "autoblks_shared:autoblkLongitudinalDriver:blkPrm_Kff"; Kg "autoblks_shared:autoblkLongitudinalDriver:blkPrm_Kg"; VehVelVec "autoblks_shared:autoblkLongitudinalDriver:blkPrm_VehVelVec"; KffVec "autoblks_shared:autoblkLongitudinalDriver:blkPrm_KffVec"; KpVec "autoblks_shared:autoblkLongitudinalDriver:blkPrm_KpVec"; KiVec "autoblks_shared:autoblkLongitudinalDriver:blkPrm_KiVec"; KgVec "autoblks_shared:autoblkLongitudinalDriver:blkPrm_KgVec"; m "autoblks_shared:autoblkLongitudinalDriver:blkPrm_m"; Kpt "autoblks_shared:autoblkLongitudinalDriver:blkPrm_Kpt"; tau "autoblks_shared:autoblkLongitudinalDriver:blkPrm_tau"; L "autoblks_shared:autoblkLongitudinalDriver:blkPrm_L"; aR "autoblks_shared:autoblkLongitudinalDriver:blkPrm_aR"; bR "autoblks_shared:autoblkLongitudinalDriver:blkPrm_bR"; cR "autoblks_shared:autoblkLongitudinalDriver:blkPrm_cR"; g "autoblks_shared:autoblkLongitudinalDriver:blkPrm_g"; vnom "autoblks_shared:autoblkLongitudinalDriver:blkPrm_vnom"; Kaw "autoblks_shared:autoblkLongitudinalDriver:blkPrm_Kaw"; tauerr "autoblks_shared:autoblkLongitudinalDriver:blkPrm_tauerr"; tauPt "autoblks_shared:autoblkLongitudinalDriver:blkPrm_tauPt"; GearInit "autoblks_shared:autoblkLongitudinalDriver:blkPrm_GearInit"; tShift "autoblks_shared:autoblkLongitudinalDriver:blkPrm_tShift"; pdlVec "autoblks_shared:autoblkLongitudinalDriver:blkPrm_pdlVec"; upShftTbl "autoblks_shared:autoblkLongitudinalDriver:blkPrm_upShftTbl"; dwnShftTbl "autoblks_shared:autoblkLongitudinalDriver:blkPrm_dwnShftTbl"; tClutch "autoblks_shared:autoblkLongitudinalDriver:blkPrm_tClutch"; tRev "autoblks_shared:autoblkLongitudinalDriver:blkPrm_tRev"; tPark "autoblks_shared:autoblkLongitudinalDriver:blkPrm_tPark"; UpGearVec "autoblks_shared:autoblkLongitudinalDriver:blkPrm_UpGearVec"; DownGearVec "autoblks_shared:autoblkLongitudinalDriver:blkPrm_DownGearVec"
      mask help: autoblks_shared:autoblkLongitudinalDriver:blkDesc
      mask init:
      | [~]=autosharedicon('autoliboperlong',gcb,0);
      mask Help: eval('autosharedhelp(''pbopmodlong'')');
      mask TypeOptions cntrlType: autoblks_shared:autoblkLongitudinalDriver:blkCmb_cntrlType_c1 | autoblks_shared:autoblkLongitudinalDriver:blkCmb_cntrlType_c2 | autoblks_shared:autoblkLongitudinalDriver:blkCmb_cntrlType_c3
      mask Callback cntrlType: [~]=autosharedicon('autoliboperlong',gcb,1);
      mask TypeOptions shftType: Longitudinal Driver/shftType
      mask Callback shftType: [~]=autosharedicon('autoliboperlong',gcb,1);
      mask TypeOptions velUnits: VelRef/Unit
      mask Callback velUnits: [~]=autosharedicon('autoliboperlong',gcb,1);
      mask DialogControl modeConfig Prompt: autoblks_shared:autoblkLongitudinalDriver:blkDlg_modeConfig
      mask DialogControl sigConfigPanel Prompt: autoblks_shared:autoblkLongitudinalDriver:blkDlg_sigConfigPanel
      mask DialogControl extAccelOvr Prompt: Accelerator override
      mask DialogControl extDecelOvr Prompt: Decelerator override
      mask DialogControl extAccelHld Prompt: Accelerator hold
      mask DialogControl extDecelHld Prompt: Decelerator hold
      mask DialogControl extAccelZero Prompt: Accelerator disable
      mask DialogControl extDecelZero Prompt: Decelerator disable
      mask DialogControl cntrlType Prompt: Control type, cntrlType:
      mask DialogControl shftType Prompt: Shift type, shftType:
      mask DialogControl velUnits Prompt: Reference and feedback units, velUnits [velUnits]:
      mask DialogControl gearOut Prompt: Output gear signal
      mask DialogControl CntrlParamPanel Prompt: autoblks_shared:autoblkLongitudinalDriver:blkDlg_CntrlParamPanel
      mask DialogControl PIParam Prompt: autoblks_shared:autoblkLongitudinalDriver:blkDlg_PIParam
      mask DialogControl Kp Prompt: Proportional gain, Kp []:
      mask DialogControl Ki Prompt: Integral gain, Ki []:
      mask DialogControl Kff Prompt: Velocity feed-forward, Kff []:
      mask DialogControl Kg Prompt: Grade angle feed-forward, Kg [1/deg]:
      mask DialogControl PISchedParam Prompt: autoblks_shared:autoblkLongitudinalDriver:blkDlg_PISchedParam
      mask DialogControl VehVelVec Prompt: Velocity gain breakpoints:
      mask DialogControl KffVec Prompt: Velocity feed-forward gain values, KffVec []:
      mask DialogControl KpVec Prompt: Proportional gain values, KpVec []:
      mask DialogControl KiVec Prompt: Integral gain values, KiVec []:
      mask DialogControl KgVec Prompt: Grade angle feed-forward values, KgVec [1/deg]:
      mask DialogControl PredParam Prompt: autoblks_shared:autoblkLongitudinalDriver:blkDlg_PredParam
      mask DialogControl m Prompt: Vehicle mass, m [kg]:
      mask DialogControl Kpt Prompt: Effective vehicle total tractive force, Kpt [N]:
      mask DialogControl tau Prompt: Driver response time, tau [s]:
      mask DialogControl L Prompt: Preview distance, L [m]:
      mask DialogControl aR Prompt: Rolling resistance coefficient, aR [N]:
      mask DialogControl bR Prompt: Rolling and driveline resistance coefficient, bR [N*s/m]:
      mask DialogControl cR Prompt: Aerodynamic drag coefficient, cR [N*s^2/m^2]:
      mask DialogControl g Prompt: Gravitational constant, g [m/s^2]:
      mask DialogControl vnom Prompt: Nominal speed, vnom [velUnits]:
      mask DialogControl Kaw Prompt: Anti-windup, Kaw []:
      mask DialogControl tauerr Prompt: Error filter time constant, tauerr [s]:
      mask DialogControl tauPt Prompt: Powertrain time constant, tauPt [s]:
      mask DialogControl shiftParamPanel Prompt: autoblks_shared:autoblkLongitudinalDriver:blkDlg_shiftParamPanel
      mask DialogControl GearInit Prompt: Initial gear, GearInit []:
      mask DialogControl tShift Prompt: Time required to shift, tShift [s]:
      mask DialogControl pdlVec Prompt: Up and down shift accelerator pedal positions, pdlVec []:
      mask DialogControl upShftTbl Prompt: Upshift velocity data table, upShftTbl [velUnits]:
      mask DialogControl dwnShftTbl Prompt: Downshift velocity data table, dwnShftTbl [velUnits]:
      mask DialogControl tClutch Prompt: Time required to shift, tClutch [s]:
      mask DialogControl tRev Prompt: Time required to engage reverse from neutral, tRev [s]:
      mask DialogControl tPark Prompt: Time required to engage park from neutral, tPark [s]:
      mask DialogControl UpGearVec Prompt: Upshift gear vector, UpGearVec []:
      mask DialogControl DownGearVec Prompt: Downshift gear vector, DownGearVec []:
      mask Display:
      | try
      |     IconInfo = autosharedicon('autoliboperlong', gcb, 4);
      | 
      |     image(IconInfo.image, IconInfo.position);
      | 
      |     for i = 1:numel(IconInfo.lconn)
      |         port_label('lconn', i, IconInfo.lconn{i})
      |     end
      | 
      |     for j = 1:numel(IconInfo.rconn)
      |         port_label('rconn', j, IconInfo.rconn{j})
      |     end
      | 
      |     for k = 1:numel(IconInfo.input)
      |         port_label('input', k, IconInfo.input{k})
      |     end
      | 
      |     for m = 1:numel(IconInfo.output)
      |         port_label('output', m, IconInfo.output{m})
      |     end
      | catch
      |     fprintf('Longitudinal \n Driver')
      | end
  Regen Braking : Subsystem
      mask Display: disp('Regen Braking')
  Terminator : Terminator
  EMTrqCmd : Outport
  VcuBrkPrsCmd : Outport  Port=2
  wires:
  Longitudinal Driver/2(AccelCmd) -> Regen Braking/2(AccelPdl)
  Regen Braking/1(EMTrqCmd) -> EMTrqCmd/1
  VehSpdFdbk/1 -> Regen Braking/4(VehSpdFdbk), Longitudinal Driver/2(VelFdbk)
  Longitudinal Driver/3(DecelCmd) -> Regen Braking/3(DecelCmd)
  VehRef/1 -> Longitudinal Driver/1(VelRef)
  EMSpd/1 -> Regen Braking/1(EMSpd)
  Regen Braking/2(VcuBrkPrsCmd) -> VcuBrkPrsCmd/1
  Constant/1 -> Longitudinal Driver/3(Grade)
  Longitudinal Driver/1(Info) -> Terminator/1

== system BEV_Thermal_Management/Controls/Fan Control ==
  p_cond : Inport
  T_env : Inport  Port=2
  cmd_comp : Inport  Port=3
  T_motor : Inport  Port=4
  Condenser Requirement : Subsystem
  Constant : Constant  Value=0
  MinMax : MinMax  Function=max  Inputs=2
  Motor Requirement : Subsystem
  Switch : Switch  Criteria=u2 > Threshold  SaturateOnIntegerOverflow=off  InputSameDT=off
  cmd_fan : Outport
  wires:
  MinMax/1 -> cmd_fan/1
  T_motor/1 -> Motor Requirement/1(T_motor)
  p_cond/1 -> Condenser Requirement/1(p_cond)
  T_env/1 -> Condenser Requirement/2(T_env)
  cmd_comp/1 -> Switch/2
  Condenser Requirement/1(cmd_fan) -> Switch/1
  Constant/1 -> Switch/3
  Switch/1 -> MinMax/1
  Motor Requirement/1(cmd_fan) -> MinMax/2

== system BEV_Thermal_Management/DCDC/PWRS7 ==
  Electrical Reference1 : fl_lib/Electrical/Electrical Elements/Electrical Reference
  Power : fl_lib/Physical Signals/Sinks/PS Terminator
  Power Sensor : ee_lib/Sensors & Transducers/Power Sensor  measurement_type=1  averaging_period=1e-4 s
  HV : PMIOPort  Side=Left
  DCDC : PMIOPort  Port=2  Side=Right
  connections:
  Power/LConn1 -- Power Sensor/RConn1
  Power Sensor/LConn2 -- DCDC/RConn1
  Electrical Reference1/LConn1 -- Power Sensor/LConn3
  Power Sensor/LConn1 -- HV/RConn1

== system BEV_Thermal_Management/DCDC/PWRS8 ==
  Electrical Reference1 : fl_lib/Electrical/Electrical Elements/Electrical Reference
  Power : fl_lib/Physical Signals/Sinks/PS Terminator
  Power Sensor : ee_lib/Sensors & Transducers/Power Sensor  measurement_type=1  averaging_period=1e-4 s
  DCDC : PMIOPort  Side=Left
  LV : PMIOPort  Port=2  Side=Right
  connections:
  Power/LConn1 -- Power Sensor/RConn1
  Power Sensor/LConn2 -- LV/RConn1
  Electrical Reference1/LConn1 -- Power Sensor/LConn3
  Power Sensor/LConn1 -- DCDC/RConn1

== system BEV_Thermal_Management/DCDC/SC8 ==
  Absolute Reference (TL) : fl_lib/Thermal Liquid/Elements/Absolute Reference (TL)
  PS-Simulink Converter1 : nesl_utility/PS-Simulink Converter  PhysicalDomain=network_engine_domain  SubClassName=ps_output  LeftPortType=input  RightPortType=output  PseudoPeriodic=off  Frequencies=[]  VectorFormat=inherit  Unit=degC  AffineConversion=on
  Pressure & Temperature Sensor (TL) : fl_lib/Thermal Liquid/Sensors/Pressure & Temperature Sensor (TL)  reference=foundation.enum.MeasurementReference.difference  pressure=true  pressure_spec=foundation.enum.PressureMeasementSpec.Absolute  temperature=true
      settings: InternalSimscapePortConfiguration="{\"Bottom\":[{\"id\":\"T\",\"label\":\"T\",\"type\":\"output\"}],\"Left\":[{\"id\":\"A\",\"label\":\"A\",\"type\":\"foundation.thermal_liquid.thermal_liquid\"}],\"Right\":[{\"id\":\"B\",\"label\":\"B\",\"type\":\"foundation.thermal_liquid.thermal_liquid\"},{\"id\":\"P\",\"label\":\"P\",\"type\":\"output\"}],\"Top\":[]}"
  Terminator : Terminator
  B : PMIOPort  Side=Left
  A : PMIOPort  Port=2  Side=Right
  wires:
  PS-Simulink Converter1/1 -> Terminator/1  "tempCoolDCOut"
  connections:
  Pressure & Temperature Sensor (TL)/LConn1 -- A/RConn1 -- B/RConn1
  Absolute Reference (TL)/LConn1 -- Pressure & Temperature Sensor (TL)/RConn1
  PS-Simulink Converter1/LConn1 -- Pressure & Temperature Sensor (TL)/RConn3

== system BEV_Thermal_Management/DCDC/SC9 ==
  Absolute Reference (TL) : fl_lib/Thermal Liquid/Elements/Absolute Reference (TL)
  PS-Simulink Converter1 : nesl_utility/PS-Simulink Converter  PhysicalDomain=network_engine_domain  SubClassName=ps_output  LeftPortType=input  RightPortType=output  PseudoPeriodic=off  Frequencies=[]  VectorFormat=inherit  Unit=degC  AffineConversion=on
  Pressure & Temperature Sensor (TL) : fl_lib/Thermal Liquid/Sensors/Pressure & Temperature Sensor (TL)  reference=foundation.enum.MeasurementReference.difference  pressure=true  pressure_spec=foundation.enum.PressureMeasementSpec.Absolute  temperature=true
      settings: InternalSimscapePortConfiguration="{\"Bottom\":[{\"id\":\"T\",\"label\":\"T\",\"type\":\"output\"}],\"Left\":[{\"id\":\"A\",\"label\":\"A\",\"type\":\"foundation.thermal_liquid.thermal_liquid\"}],\"Right\":[{\"id\":\"B\",\"label\":\"B\",\"type\":\"foundation.thermal_liquid.thermal_liquid\"},{\"id\":\"P\",\"label\":\"P\",\"type\":\"output\"}],\"Top\":[]}"
  Terminator : Terminator
  B : PMIOPort  Side=Left
  A : PMIOPort  Port=2  Side=Right
  wires:
  PS-Simulink Converter1/1 -> Terminator/1  "tempCoolDCIn"
  connections:
  Pressure & Temperature Sensor (TL)/LConn1 -- A/RConn1 -- B/RConn1
  Absolute Reference (TL)/LConn1 -- Pressure & Temperature Sensor (TL)/RConn1
  PS-Simulink Converter1/LConn1 -- Pressure & Temperature Sensor (TL)/RConn3

== system BEV_Thermal_Management/Driveline/PWRS6 ==
  Ideal Force Sensor : fl_lib/Mechanical/Mechanical Sensors/Ideal Force Sensor
  Ideal Translational Motion Sensor : fl_lib/Mechanical/Mechanical Sensors/Ideal Translational Motion Sensor  reference=foundation.enum.MeasurementReference.difference  acceleration_port=false  velocity_port=true  position_port=false  offset=0 m
      settings: InternalSimscapePortConfiguration="{\"Bottom\":[],\"Left\":[{\"id\":\"R\",\"label\":\"R\",\"type\":\"foundation.mechanical.translational.translational\"}],\"Right\":[{\"id\":\"C\",\"label\":\"C\",\"type\":\"foundation.mechanical.translational.translational\"},{\"id\":\"V\",\"label\":\"V\",\"type\":\"output\"}],\"Top\":[]}"
  Mechanical Translational Reference : fl_lib/Mechanical/Translational Elements/Mechanical Translational Reference
  PS Terminator : fl_lib/Physical Signals/Sinks/PS Terminator
  Power : fl_lib/Physical Signals/Functions/PS Product
  V : PMIOPort  Side=Left
  W : PMIOPort  Port=2  Side=Right
  connections:
  V/RConn1 -- Ideal Force Sensor/RConn1
  PS Terminator/LConn1 -- Power/RConn1
  Mechanical Translational Reference/LConn1 -- Ideal Translational Motion Sensor/RConn1
  W/RConn1 -- Ideal Translational Motion Sensor/LConn1 -- Ideal Force Sensor/LConn1
  Power/LConn2 -- Ideal Force Sensor/RConn2
  Power/LConn1 -- Ideal Translational Motion Sensor/RConn2

== system BEV_Thermal_Management/Driveline/Passenger mass ==
  Bias : Bias  Bias=-1  SaturateOnIntegerOverflow=off
  Gain1 : Gain  Gain=75
  Out1 : Outport
  wires:
  Bias/1 -> Gain1/1
  Gain1/1 -> Out1/1
  [N_occupant] -> Bias/1
